simulink model "Simulink_Simulation"  (R2025a)
settings: Solver=VariableStepAuto  StartTime=0.0  StopTime=100.0  RelTol=1e-3
values from neighbouring files (symbols this model uses):
  M = M_values(m)    [MatLab_Code.m]    (also in Simulink_Code.m = 8)
libraries: commsink2 x2, simulink x2, commdigbbndam3 x2, commchan3 x1, commdigbbndpm3 x1, dspsigops x1, commrandsrc3 x1
settings Model: Creator=Youssef Zaher  LastModifiedBy=Pioneer

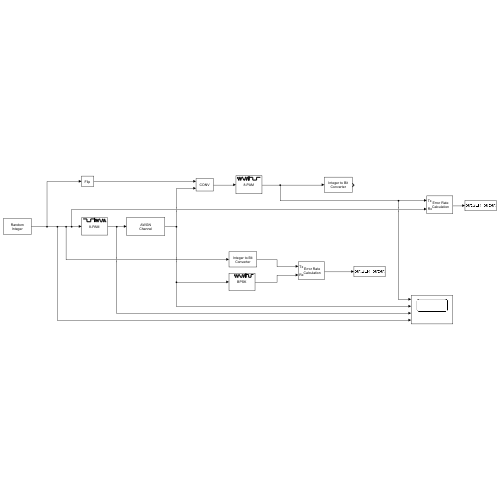
[thumbnail: Simulink's stored preview of the top-level diagram]
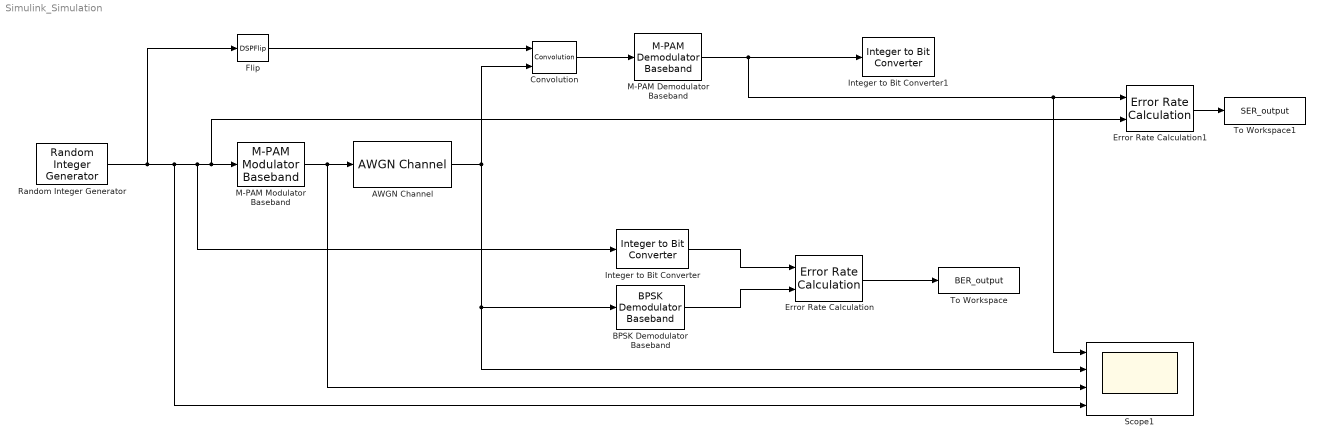
== system Simulink_Simulation ==
  AWGN Channel : commchan3/AWGN Channel  LegacyMode=off  NoiseMethod="Signal to noise ratio  (SNR)"  noiseMode="Signal to noise ratio  (SNR)"  EbNo=snr_db  EsNo=10  SNR=snr_db  BitsPerSymbol=log2(M)  SignalPower=1  SpecifySymbolPeriod=off  SamplesPerSymbol=1  SymbolPeriod=1  VarianceSource=Parameter  Variance=1  RandomStream=Global stream  Seed=67  SimulateUsing=Code generation
  BPSK Demodulator Baseband : commdigbbndpm3/BPSK Demodulator Baseband  DecType=Hard decision  VarSource=Dialog  Variance=1  Ph=0  outDtype=Inherit via internal rule  derotateFactorWordLen=16  derotateFactorDataTypeStr=Inherit: Same word length as input  derotateFactorLastDataTypeStr=Inherit: Same word length as input
  Convolution : dspsigops/Convolution  domain=Time  roundingMode=Floor  overflowMode=off  outputDataTypeStr=Inherit: Same as accumulator  outputMin=[]  outputMax=[]  outputLastDataTypeStr=Inherit: Same as accumulator
  Error Rate Calculation : commsink2/Error Rate Calculation  N=0  st_delay=0  cp_mode=Entire frame  subframe=[]  PMode=Port  WsName=ErrorVec  RsMode2=off  stop=off  numErr=100  maxBits=1e6
  Error Rate Calculation1 : commsink2/Error Rate Calculation  N=0  st_delay=0  cp_mode=Entire frame  subframe=[]  PMode=Port  WsName=ErrorVec  RsMode2=off  stop=off  numErr=100  maxBits=1e6
  Flip : DSPFlip
  Integer to Bit Converter : simulink/Logic and Bit Operations/Integer to Bit Converter  nbits=log2(M)  signedInputValues=Unsigned  bitOrder=MSB first  outDtype=double
  Integer to Bit Converter1 : simulink/Logic and Bit Operations/Integer to Bit Converter  nbits=log2(M)  signedInputValues=Unsigned  bitOrder=MSB first  outDtype=double
  M-PAM Demodulator Baseband : commdigbbndam3/M-PAM Demodulator Baseband  M=M  OutType=Integer  Dec=Gray  PowType=Average Power  MinDist=1  AvgPow=1  PeakPow=1  outDtype1=Inherit via internal rule  outDtype2=Inherit via internal rule  denormFactorWordLen=16  denormFactorDataTypeStr=Inherit: Same word length as input  denormFactorLastDataTypeStr=Inherit: Same word length as input  prodOutWordLen=16  prodOutRoundingMode=Floor  prodOutOverflowMode=Wrap  prodOutOvFlMode=off  prodOutOvFlModeLastStrValue=off  sumWordLen=16
  M-PAM Modulator Baseband : commdigbbndam3/M-PAM Modulator Baseband  M=M  InType=Integer  Enc=Gray  PowType=Average Power  MinDist=1  AvgPow=1  PeakPow=1  outDtype=double  outWordLen=16  outUDDataType=sfix(16)  outFracLenMode=Best precision  outFracLen=15  outDataTypeStr=double  outLastDataTypeStr=double
  Random Integer Generator : commrandsrc3/Random Integer Generator  SetSize=M  SeedSource=Auto  Seed=0  SampleTime=1  SamplesPerFrame=1  OutputDataType=double  SimulateUsing=Interpreted execution
  Scope1 : Scope  NumInputPorts=4
      settings: ActiveDisplayYMinimum=-1  ActiveDisplayYMaximum=1
  To Workspace : ToWorkspace  VariableName=BER_output  SampleTime=-1
  To Workspace1 : ToWorkspace  VariableName=SER_output  SampleTime=-1
  wires:
  M-PAM Modulator Baseband/1 -> Scope1/3, AWGN Channel/1
  Error Rate Calculation/1 -> To Workspace/1
  M-PAM Demodulator Baseband/1 -> Scope1/1, Error Rate Calculation1/1, Integer to Bit Converter1/1
  Integer to Bit Converter/1 -> Error Rate Calculation/1
  Error Rate Calculation1/1 -> To Workspace1/1
  AWGN Channel/1 -> Scope1/2, BPSK Demodulator Baseband/1, Convolution/2
  BPSK Demodulator Baseband/1 -> Error Rate Calculation/2
  Convolution/1 -> M-PAM Demodulator Baseband/1
  Random Integer Generator/1 -> Flip/1, Error Rate Calculation1/2, M-PAM Modulator Baseband/1, Integer to Bit Converter/1, Scope1/4
  Flip/1 -> Convolution/1
